simulink model "RobustFormationControl_IntegerModel"  (R2023a)
settings: Solver=ode3  StartTime=0.0  StopTime=30  FixedStep=0.0001  RelTol=1e-3
InitFcn:
  | % % Parameters for the fractional order NTFSMC:
  | % Sliding Surface " Sx, Sy, and Sz ":
  | %------------------------
  | % 10
  | % 10
  | cx = 2*[4 4 4];
  | cxx = 1*[0.01 0.01 0.01];
  | 
  | cx1 = cx(1);
  | cy1 = cx(2);
  | cz1 = cx(3);
  | 
  | cx2 = cxx(1);
  | cy2 = cxx(2);
  | cz2 = cxx(3);
  | 
  | alpha1 = [0.6 0.6 0.6];
  | alpha2 = [0.1 0.1 0.1];
  | 
  | gammaX = [3 3 3];
  | gx  = gammaX(1);
  | gy = gammaX(2);
  | gz = gammaX(3);
  | 
  | p = 10;
  | q = 10;
  | 
  | % Sliding Surface " S_Phi , S_Theta, and  S_Psi":
  | %------------------------
  | cP = 2*[4 4 4];
  | cPP = 1*[0.01 0.01 0.01 0.01];
  | 
  | cPhi1 = cP(1);
  | cTheta1 = cP(2);
  | cPsi1 = cP(3);
  | 
  | cPhi2 = cPP(1);
  | cTheta2 = cPP(2);
  | cPsi2 = cPP(3);
  | gammaP = [3 3 3];
  | 
  | %=========================
  | %=========================
  | SigmaX = 1*[0.01 0.01 0.01];
  | SigmaXX =1*[1 1 1];
  | 
  | Sigma1X = SigmaX(1);
  | Sigma1Y = SigmaX(2);
  | Sigma1Z = SigmaX(3);
  | %-----
  | Sigma2X = SigmaXX(1);
  | Sigma2Y = SigmaXX(2);
  | Sigma2Z = SigmaXX(3);
  | 
  | 
  | SigmaP = 1*[0.01 0.01 0.01];
  | SigmaPP =1*[1 1 1];
  | 
  | Sigma1Phi   = SigmaP(1);
  | Sigma1Theta = SigmaP(2);
  | ... (+80 lines)
values from neighbouring files (symbols this model uses):
  a1 = (Iyy - Izz)/Ixx    (= -0.812397034596)    [init_quadrotor_params.m]
  a2 = (Izz - Ixx)/Iyy    (= 0.812397034596)    [init_quadrotor_params.m]
  a3 = (Ixx - Iyy)/Izz    (= 0)    [init_quadrotor_params.m]
  a4 = - Ktx/m    (= -0.00114547325103)    [init_quadrotor_params.m]
  a5 = - Kty/m    (= -0.00114547325103)    [init_quadrotor_params.m]
  a6 = - Ktz/m    (= -0.00130740740741)    [init_quadrotor_params.m]
  b = 2.980e-5    (= 2.98e-05)    [init_quadrotor_params.m]
  b1 = - Jr/Ixx    (= -0.00584534596376)    [init_quadrotor_params.m]
  b2 = Jr/Iyy    (= 0.00584534596376)    [init_quadrotor_params.m]
  b3 = - Kfz/Izz    (= -0.0721963413248)    [init_quadrotor_params.m]
  b4 = 1/m    (= 2.05761316872)    [init_quadrotor_params.m]
  b5 = 1/m    (= 2.05761316872)    [init_quadrotor_params.m]
  b6 = 1/m    (= 2.05761316872)    [init_quadrotor_params.m]
  c1 = - Kfx/Ixx    (= -0.114641680395)    [init_quadrotor_params.m]
  c2 = - Kfy/Iyy    (= -0.114641680395)    [init_quadrotor_params.m]
  c3 = 1/Izz    (= 113.62345188)    [init_quadrotor_params.m]
  d = 1.12e-06    [init_quadrotor_params.m]
  d1 = L/Ixx    (= 46.334431631)    [init_quadrotor_params.m]
  d2 = L/Iyy    (= 46.334431631)    [init_quadrotor_params.m]
  g = 9.81    [init_quadrotor_params.m]
  Ixx = 4.856e-3    (= 0.004856)    [init_quadrotor_params.m]
  Iyy = 4.856e-3    (= 0.004856)    [init_quadrotor_params.m]
  Izz = 8.801e-3    (= 0.008801)    [init_quadrotor_params.m]
  Jr = 2.8385e-5    (= 2.8385e-05)    [init_quadrotor_params.m]
  Kfx = 5.567e-4    (= 0.0005567)    [init_quadrotor_params.m]
  Kfy = 5.567e-4    (= 0.0005567)    [init_quadrotor_params.m]
  Kfz = 6.354e-4    (= 0.0006354)    [init_quadrotor_params.m]
  Ktx = 5.5670e-4    (= 0.0005567)    [init_quadrotor_params.m]
  Kty = 5.5670e-4    (= 0.0005567)    [init_quadrotor_params.m]
  Ktz = 6.3540e-4    (= 0.0006354)    [init_quadrotor_params.m]
  L = 0.225    [init_quadrotor_params.m]
  m = 0.486    [init_quadrotor_params.m]
libraries: fod x120, eeStairGenerator x5
(part 4 of 9)

== system RobustFormationControl_IntegerModel/Integer Leader and four followers/Follower 1 System/Follower 1 Quadrotor Model/Quadrotor Dynamic System/Rotational System ==
  U2 : Inport
  U3 : Inport  Port=2
  U4 : Inport  Port=3
  Omega : Inport  Port=4
  Equation1 : Subsystem
  Equation2 : Subsystem
  Equation3 : Subsystem
  Phi or x1 : Outport  VectorParamsAs1DForOutWhenUnconnected=off
  Theta or x3 : Outport  Port=2  VectorParamsAs1DForOutWhenUnconnected=off
  Psi or x5 : Outport  Port=3  VectorParamsAs1DForOutWhenUnconnected=off
  x2 : Outport  Port=4  VectorParamsAs1DForOutWhenUnconnected=off
  x4 : Outport  Port=5  VectorParamsAs1DForOutWhenUnconnected=off
  x6 : Outport  Port=6  VectorParamsAs1DForOutWhenUnconnected=off
  wires:
  Equation1/1(x1 = Phi) -> Phi or x1/1
  Equation3/1(x5 =Psi) -> Psi or x5/1
  U2/1 -> Equation1/3(U2)
  U3/1 -> Equation2/3(U3)
  Equation3/2(x6) -> Equation2/2(x6), x6/1, Equation1/2(x6)
  Equation2/1(x3 =Theta) -> Theta or x3/1
  U4/1 -> Equation3/3(U4)
  Omega/1 -> Equation2/4(Omega), Equation1/4(Omega)
  Equation1/2(x2) -> x2/1, Equation2/1(x2), Equation3/1(x2)
  Equation2/2(x4) -> x4/1, Equation3/2(x4), Equation1/1(x4)

== system RobustFormationControl_IntegerModel/Integer Leader and four followers/Follower 1 System/Follower 1 Quadrotor Model/Quadrotor Dynamic System/Translational System ==
  U1 : Inport
  Ux : Inport  Port=2
  Uy : Inport  Port=3
  x1 : Inport  Port=4
  x3 : Inport  Port=5
  Equation4 : Subsystem
  Equation5 : Subsystem
  Equation6 : Subsystem
  x or x7 : Outport  VectorParamsAs1DForOutWhenUnconnected=off
  y or x9 : Outport  Port=2  VectorParamsAs1DForOutWhenUnconnected=off
  z or x11 : Outport  Port=3  VectorParamsAs1DForOutWhenUnconnected=off
  xdot or x8 : Outport  Port=4  VectorParamsAs1DForOutWhenUnconnected=off
  ydot or x10 : Outport  Port=5  VectorParamsAs1DForOutWhenUnconnected=off
  zdot or x12 : Outport  Port=6  VectorParamsAs1DForOutWhenUnconnected=off
  wires:
  Ux/1 -> Equation4/2(Ux)
  Uy/1 -> Equation5/2(Uy)
  x1/1 -> Equation6/2(x1)
  x3/1 -> Equation6/3(x3)
  Equation5/1(x9 = y) -> y or x9/1
  Equation6/1(x11 = z) -> z or x11/1
  Equation4/1(x7 = x) -> x or x7/1
  U1/1 -> Equation6/1(U1), Equation5/1(U1), Equation4/1(U1)
  Equation4/2(x8 = xdot) -> xdot or x8/1
  Equation5/2(x10 = ydot) -> ydot or x10/1
  Equation6/2(x12 = zdot) -> zdot or x12/1

== system RobustFormationControl_IntegerModel/Integer Leader and four followers/Follower 2 System/Follower 2 Quadrotor Model/Control Module1/Desired System ==
  Phi_d : Inport
  Theta_d : Inport  Port=2
  Psi_d : Inport  Port=3
  xd : Inport  Port=4
  yd : Inport  Port=5
  zd : Inport  Port=6
  Derivative{,1..5} (6 alike) : Derivative
  xd1 : Outport  VectorParamsAs1DForOutWhenUnconnected=off
  xd2 : Outport  Port=2  VectorParamsAs1DForOutWhenUnconnected=off
  xd3 : Outport  Port=3  VectorParamsAs1DForOutWhenUnconnected=off
  xd4 : Outport  Port=4  VectorParamsAs1DForOutWhenUnconnected=off
  xd5 : Outport  Port=5  VectorParamsAs1DForOutWhenUnconnected=off
  xd6 : Outport  Port=6  VectorParamsAs1DForOutWhenUnconnected=off
  xd7 : Outport  Port=7  VectorParamsAs1DForOutWhenUnconnected=off
  xd8 : Outport  Port=8  VectorParamsAs1DForOutWhenUnconnected=off
  xd9 : Outport  Port=9  VectorParamsAs1DForOutWhenUnconnected=off
  xd10 : Outport  Port=10  VectorParamsAs1DForOutWhenUnconnected=off
  xd11 : Outport  Port=11  VectorParamsAs1DForOutWhenUnconnected=off
  xd12 : Outport  Port=12  VectorParamsAs1DForOutWhenUnconnected=off
  wires:
  Phi_d/1 -> Derivative/1, xd1/1
  Derivative/1 -> xd2/1
  Derivative1/1 -> xd4/1
  Theta_d/1 -> Derivative1/1, xd3/1
  Psi_d/1 -> Derivative2/1, xd5/1
  Derivative2/1 -> xd6/1
  Derivative3/1 -> xd8/1
  Derivative4/1 -> xd10/1
  Derivative5/1 -> xd12/1
  xd/1 -> Derivative3/1, xd7/1
  yd/1 -> Derivative4/1, xd9/1
  zd/1 -> Derivative5/1, xd11/1

== system RobustFormationControl_IntegerModel/Integer Leader and four followers/Follower 2 System/Follower 2 Quadrotor Model/Control Module1/Omega Equations ==
  U1 : Inport
  U2 : Inport  Port=2
  U3 : Inport  Port=3
  U4 : Inport  Port=4
  Add1 : Sum  Inputs=+--
  Add2 : Sum  Inputs=+++
  Add3 : Sum  Inputs=++-
  Add5 : Sum  Inputs=+-+
  Control Inputs : Subsystem
  Gain11 : Gain  Gain=1/(4*b)
  Gain12 : Gain  Gain=1/(4*d)
  Gain7 : Gain  Gain=1/(2*b)
  Gain8 : Gain  Gain=1/(2*b)
  Omega : Outport  VectorParamsAs1DForOutWhenUnconnected=off
  wires:
  Add5/1 -> Control Inputs/1(w1_sqt)
  Add1/1 -> Control Inputs/2(w2_sqt)
  Add2/1 -> Control Inputs/3(w3_sqt)
  Gain11/1 -> Add5/1, Add3/1, Add2/1, Add1/1
  Gain12/1 -> Add5/3, Add2/3, Add3/3, Add1/3
  Gain7/1 -> Add5/2, Add2/2
  Gain8/1 -> Add3/2, Add1/2
  U4/1 -> Gain12/1
  U1/1 -> Gain11/1
  U3/1 -> Gain7/1
  U2/1 -> Gain8/1
  Add3/1 -> Control Inputs/4(w4_sqt)
  Control Inputs/1(Omega) -> Omega/1

== system RobustFormationControl_IntegerModel/Integer Leader and four followers/Follower 2 System/Follower 2 Quadrotor Model/Control Module1/Subsystem ==
  Ux : Inport
  Uy : Inport  Port=2
  Psi_d : Inport  Port=3
  Subsystem : Subsystem
  Subsystem1 : Subsystem
  Phi_d : Outport  VectorParamsAs1DForOutWhenUnconnected=off
  Theta_d : Outport  Port=2  VectorParamsAs1DForOutWhenUnconnected=off
  wires:
  Ux/1 -> Subsystem1/1(Ux), Subsystem/1(Ux)
  Uy/1 -> Subsystem1/2(Uy), Subsystem/2(Uy)
  Psi_d/1 -> Subsystem1/3(Psi_d), Subsystem/3(Psi_d)
  Subsystem/1(Phi_d) -> Subsystem1/4(Phi_d), Phi_d/1
  Subsystem1/1(Theta_d) -> Theta_d/1

== system RobustFormationControl_IntegerModel/Integer Leader and four followers/Follower 2 System/Follower 2 Quadrotor Model/Control Module1/Subsystem1 ==
  x1 : Inport
  x2 : Inport  Port=2
  x3 : Inport  Port=3
  x4 : Inport  Port=4
  x5 : Inport  Port=5
  x6 : Inport  Port=6
  x7 : Inport  Port=7
  x8 : Inport  Port=8
  x9 : Inport  Port=9
  x10 : Inport  Port=10
  x11 : Inport  Port=11
  x12 : Inport  Port=12
  xd1 : Inport  Port=13
  xd2 : Inport  Port=14
  xd3 : Inport  Port=15
  xd4 : Inport  Port=16
  xd5 : Inport  Port=17
  xd6 : Inport  Port=18
  xL : Inport  Port=19
  dX : Inport  Port=20
  yL : Inport  Port=21
  dY : Inport  Port=22
  zL : Inport  Port=23
  dZ : Inport  Port=24
  Subsystem : Subsystem
  Subsystem1 : Subsystem
  Subsystem2 : Subsystem
  Subsystem3 : Subsystem
  Subsystem4 : Subsystem
  Subsystem6 : Subsystem
  S2 : Outport  VectorParamsAs1DForOutWhenUnconnected=off
  S4 : Outport  Port=2  VectorParamsAs1DForOutWhenUnconnected=off
  S6 : Outport  Port=3  VectorParamsAs1DForOutWhenUnconnected=off
  S8 : Outport  Port=4  VectorParamsAs1DForOutWhenUnconnected=off
  S10 : Outport  Port=5  VectorParamsAs1DForOutWhenUnconnected=off
  S12 : Outport  Port=6  VectorParamsAs1DForOutWhenUnconnected=off
  wires:
  x1/1 -> [x1]
  x2/1 -> [x2]
  x3/1 -> [x3]
  x4/1 -> [x4]
  x5/1 -> [x5]
  x6/1 -> [x6]
  x7/1 -> [x7]
  x8/1 -> [x8]
  x9/1 -> [x9]
  x10/1 -> [x10]
  x11/1 -> [x11]
  x12/1 -> [x12]
  xd1/1 -> [xd1]
  dY/1 -> [dY]
  xd2/1 -> [xd2]
  xd3/1 -> [xd3]
  xd4/1 -> [xd4]
  xd5/1 -> [xd5]
  xd6/1 -> [xd6]
  xL/1 -> [xL]
  dX/1 -> [dX]
  yL/1 -> [yL]
  zL/1 -> [zL]
  dZ/1 -> [dZ]
  [x1] -> Subsystem/1(x1)
  [xd1] -> Subsystem/2(xd1)
  [x2] -> Subsystem/3(x2)
  [xd2] -> Subsystem/4(xd2)
  Subsystem/1(S2) -> S2/1
  [xd4] -> Subsystem6/4(xd4)
  [x3] -> Subsystem6/1(x3)
  [x4] -> Subsystem6/3(x4)
  [xd3] -> Subsystem6/2(xd3)
  [xd6] -> Subsystem1/4(xd6)
  [x5] -> Subsystem1/1(x5)
  [x6] -> Subsystem1/3(x6)
  [xd5] -> Subsystem1/2(xd5)
  Subsystem6/1(S4) -> S4/1
  Subsystem1/1(S6) -> S6/1
  [x9] -> Subsystem2/2(x9)
  [x10] -> Subsystem2/3(x10)
  [yL] -> Subsystem2/1(yL)
  [dY] -> Subsystem2/4(dY)
  Subsystem2/1(S10) -> S10/1
  [zL] -> Subsystem4/1(zL)
  [x8] -> Subsystem3/3(x8)
  Subsystem4/1(S12) -> S12/1
  [x12] -> Subsystem4/3(x12)
  Subsystem3/1(S8) -> S8/1
  [dZ] -> Subsystem4/4(dZ)
  [x11] -> Subsystem4/2(x11)
  [x7] -> Subsystem3/2(x7)
  [dX] -> Subsystem3/4(dX)
  [xL] -> Subsystem3/1(xL)

== system RobustFormationControl_IntegerModel/Integer Leader and four followers/Follower 2 System/Follower 2 Quadrotor Model/Control Module1/Subsystem10 ==
  x1 : Inport
  x3 : Inport  Port=2
  x11 : Inport  Port=3
  x12 : Inport  Port=4
  zL : Inport  Port=5
  dZ : Inport  Port=6
  S12 : Inport  Port=7
  Constant1 : Constant
  Divide1 : Product  Inputs=*/
  Divide2 : Product  Inputs=**  RndMeth=Zero  SaturateOnIntegerOverflow=on
  Gain : Gain  Commented=on  Gain=b6
  Product1 : Product
  Product2 : Product
  Subsystem : Subsystem
  Subsystem1 : Subsystem
  Subsystem2 : Subsystem
  Sum2 : Sum  Inputs=+++
  Trigonometric Function1 : Trigonometry  Operator=cos
  Trigonometric Function2 : Trigonometry  Operator=cos
  U1 : Outport  VectorParamsAs1DForOutWhenUnconnected=off
  wires:
  S12/1 -> [S12]
  dZ/1 -> [dZ]
  zL/1 -> [zL]
  x3/1 -> [x3]
  Sum2/1 -> Product2/2
  Product2/1 -> U1/1
  x11/1 -> [x11]
  x12/1 -> [x12]
  x1/1 -> [x1]
  [x11] -> Subsystem/2(x11)
  [x12] -> Subsystem1/1(x12)
  [zL] -> Subsystem1/2(zL)
  [zL] -> Subsystem/1(zL)
  [dZ] -> Subsystem/4(dZ)
  [x12] -> Subsystem/3(x12)
  [S12] -> Subsystem/5(S12)
  [x11] -> Subsystem2/2(x11)
  [S12] -> Subsystem2/5(S12)
  [x12] -> Subsystem2/3(x12)
  [zL] -> Subsystem2/1(zL)
  [dZ] -> Subsystem2/4(dZ)
  Subsystem/1(D2) -> Sum2/2
  Subsystem2/1(D3) -> Sum2/3
  Subsystem1/1(D1) -> Sum2/1
  Divide1/1 -> Product2/1
  Constant1/1 -> Divide1/1
  Trigonometric Function2/1 -> Product1/2
  Trigonometric Function1/1 -> Product1/1
  Divide2/1 -> Divide1/2
  Product1/1 -> Divide2/2
  [x1] -> Trigonometric Function1/1
  [x3] -> Trigonometric Function2/1
  [b6D] -> Divide2/1
  [dZ] -> Subsystem1/3(dZ)

== system RobustFormationControl_IntegerModel/Integer Leader and four followers/Follower 2 System/Follower 2 Quadrotor Model/Control Module1/Subsystem2 ==
  U1 : Inport
  x9 : Inport  Port=2
  x10 : Inport  Port=3
  yL : Inport  Port=4
  dY : Inport  Port=5
  S10 : Inport  Port=6
  Constant1 : Constant
  Divide1 : Product  Inputs=*/
  Divide2 : Product  Inputs=**  RndMeth=Zero  SaturateOnIntegerOverflow=on
  Gain1 : Gain  Commented=on  Gain=b4
  Product2 : Product
  Subsystem3 : Subsystem
  Subsystem4 : Subsystem
  Subsystem5 : Subsystem
  Sum1 : Sum  Inputs=+++
  Uy : Outport  VectorParamsAs1DForOutWhenUnconnected=off
  wires:
  S10/1 -> [S10]
  dY/1 -> [dY]
  yL/1 -> [yL]
  Product2/1 -> Uy/1
  x9/1 -> [x9]
  x10/1 -> [x10]
  U1/1 -> [U1]
  Divide1/1 -> Product2/1
  Constant1/1 -> Divide1/1
  [b5D] -> Divide2/1
  [U1] -> Divide2/2
  Divide2/1 -> Divide1/2
  [dY] -> Subsystem4/3(dY)
  [dY] -> Subsystem3/4(dY)
  Subsystem4/1(D1) -> Sum1/1
  Subsystem5/1(D3) -> Sum1/3
  [yL] -> Subsystem5/1(yL)
  Subsystem3/1(D2) -> Sum1/2
  [dY] -> Subsystem5/4(dY)
  [x9] -> Subsystem3/2(x9)
  [yL] -> Subsystem3/1(yL)
  [yL] -> Subsystem4/2(yL)
  [S10] -> Subsystem3/5(S10)
  [x9] -> Subsystem5/2(x9)
  [x10] -> Subsystem5/3(x10)
  [x10] -> Subsystem4/1(x10)
  [x10] -> Subsystem3/3(x10)
  [S10] -> Subsystem5/5(S10)
  Sum1/1 -> Product2/2

== system RobustFormationControl_IntegerModel/Integer Leader and four followers/Follower 2 System/Follower 2 Quadrotor Model/Control Module1/Subsystem4 ==
  x1 : Inport
  x2 : Inport  Port=2
  x4 : Inport  Port=3
  x6 : Inport  Port=4
  xd1 : Inport  Port=5
  xd2 : Inport  Port=6
  S2 : Inport  Port=7
  Omega : Inport  Port=8
  Constant : Constant
  Constant3 : Constant  Value=d1
  Derivative : Derivative
  Divide : Product  Inputs=*/
  Product2 : Product
  Subsystem : Subsystem
  Subsystem1 : Subsystem
  Subsystem2 : Subsystem
  Sum2 : Sum  Inputs=+++
  U2 : Outport  VectorParamsAs1DForOutWhenUnconnected=off
  wires:
  Constant/1 -> Divide/1
  Constant3/1 -> Divide/2
  S2/1 -> [S2]
  xd2/1 -> [xd2], Derivative/1
  Derivative/1 -> [xdDot2]
  xd1/1 -> [xd1]
  x2/1 -> [x2]
  Sum2/1 -> Product2/2
  Divide/1 -> Product2/1
  Product2/1 -> U2/1
  x4/1 -> [x4]
  x6/1 -> [x6]
  x1/1 -> [x1]
  [x1] -> Subsystem/1(x1)
  [x4] -> Subsystem1/1(x4)
  [x6] -> Subsystem1/2(x6)
  [x2] -> Subsystem1/3(x2)
  Omega/1 -> Subsystem1/4(Omega)
  [xdDot2] -> Subsystem1/5(xd2)
  [xd1] -> Subsystem/2(xd1)
  [xd2] -> Subsystem/4(xd2)
  [x2] -> Subsystem/3(x2)
  [S2] -> Subsystem/5(S2)
  [xd1] -> Subsystem2/2(xd1)
  [S2] -> Subsystem2/5(S2)
  [x2] -> Subsystem2/3(x2)
  [x1] -> Subsystem2/1(x1)
  [xd2] -> Subsystem2/4(xd2)
  Subsystem1/1(D1) -> Sum2/1
  Subsystem/1(D2) -> Sum2/2
  Subsystem2/1(D3) -> Sum2/3

== system RobustFormationControl_IntegerModel/Integer Leader and four followers/Follower 2 System/Follower 2 Quadrotor Model/Control Module1/Subsystem5 ==
  x5 : Inport
  x2 : Inport  Port=2
  x4 : Inport  Port=3
  x6 : Inport  Port=4
  xd5 : Inport  Port=5
  xd6 : Inport  Port=6
  S6 : Inport  Port=7
  Constant : Constant
  Constant3 : Constant  Value=c3
  Derivative : Derivative
  Divide : Product  Inputs=*/
  Product2 : Product
  Subsystem : Subsystem
  Subsystem1 : Subsystem
  Subsystem2 : Subsystem
  Sum2 : Sum  Inputs=+++
  U4 : Outport  VectorParamsAs1DForOutWhenUnconnected=off
  wires:
  Constant/1 -> Divide/1
  Constant3/1 -> Divide/2
  S6/1 -> [S6]
  xd6/1 -> [xd6], Derivative/1
  Derivative/1 -> [xdDot6]
  xd5/1 -> [xd5]
  x2/1 -> [x2]
  Sum2/1 -> Product2/2
  Divide/1 -> Product2/1
  Product2/1 -> U4/1
  x4/1 -> [x4]
  x6/1 -> [x6]
  x5/1 -> [x5]
  [x5] -> Subsystem/1(x5)
  [x4] -> Subsystem1/1(x4)
  [x6] -> Subsystem1/2(x6)
  [x2] -> Subsystem1/3(x2)
  [xdDot6] -> Subsystem1/4(xd6)
  [xd5] -> Subsystem/2(xd5)
  [xd6] -> Subsystem/4(xd6)
  [x6] -> Subsystem/3(x6)
  [S6] -> Subsystem/5(S4)
  [xd5] -> Subsystem2/2(xd5)
  [S6] -> Subsystem2/5(S6)
  [x6] -> Subsystem2/3(x6)
  [x5] -> Subsystem2/1(x5)
  [xd6] -> Subsystem2/4(xd6)
  Subsystem/1(D2) -> Sum2/2
  Subsystem2/1(D3) -> Sum2/3
  Subsystem1/1(D1) -> Sum2/1

== system RobustFormationControl_IntegerModel/Integer Leader and four followers/Follower 2 System/Follower 2 Quadrotor Model/Control Module1/Subsystem6 ==
  U1 : Inport
  x7 : Inport  Port=2
  x8 : Inport  Port=3
  xL : Inport  Port=4
  dX : Inport  Port=5
  S8 : Inport  Port=6
  Constant1 : Constant
  Divide1 : Product  Inputs=*/
  Divide2 : Product  Inputs=**  RndMeth=Zero  SaturateOnIntegerOverflow=on
  Gain1 : Gain  Commented=on  Gain=b4
  Product2 : Product
  Subsystem3 : Subsystem
  Subsystem4 : Subsystem
  Subsystem5 : Subsystem
  Sum1 : Sum  Inputs=+++
  Ux : Outport  VectorParamsAs1DForOutWhenUnconnected=off
  wires:
  S8/1 -> [S8]
  dX/1 -> [dX]
  xL/1 -> [xL]
  Product2/1 -> Ux/1
  x7/1 -> [x7]
  x8/1 -> [x8]
  U1/1 -> [U1]
  Divide1/1 -> Product2/1
  Constant1/1 -> Divide1/1
  [b4D] -> Divide2/1
  [U1] -> Divide2/2
  Divide2/1 -> Divide1/2
  [dX] -> Subsystem4/3(dX)
  [dX] -> Subsystem3/4(dX)
  Subsystem4/1(D1) -> Sum1/1
  Subsystem5/1(D3) -> Sum1/3
  [xL] -> Subsystem5/1(xL)
  Subsystem3/1(D2) -> Sum1/2
  [dX] -> Subsystem5/4(dX)
  [x7] -> Subsystem3/2(x7)
  [xL] -> Subsystem3/1(xL)
  [xL] -> Subsystem4/2(xL)
  [S8] -> Subsystem3/5(S8)
  [x7] -> Subsystem5/2(x7)
  [x8] -> Subsystem5/3(x8)
  [x8] -> Subsystem4/1(x8)
  [x8] -> Subsystem3/3(x8)
  [S8] -> Subsystem5/5(S8)
  Sum1/1 -> Product2/2

== system RobustFormationControl_IntegerModel/Integer Leader and four followers/Follower 2 System/Follower 2 Quadrotor Model/Control Module1/Subsystem8 ==
  x3 : Inport
  x2 : Inport  Port=2
  x4 : Inport  Port=3
  x6 : Inport  Port=4
  xd3 : Inport  Port=5
  xd4 : Inport  Port=6
  S4 : Inport  Port=7
  Omega : Inport  Port=8
  Constant : Constant
  Constant3 : Constant  Value=d2
  Derivative : Derivative
  Divide : Product  Inputs=*/
  Product2 : Product
  Subsystem : Subsystem
  Subsystem1 : Subsystem
  Subsystem2 : Subsystem
  Sum2 : Sum  Inputs=+++
  U3 : Outport  VectorParamsAs1DForOutWhenUnconnected=off
  wires:
  Constant/1 -> Divide/1
  Constant3/1 -> Divide/2
  S4/1 -> [S4]
  xd4/1 -> [xd4], Derivative/1
  Derivative/1 -> [xdDot4]
  xd3/1 -> [xd3]
  x2/1 -> [x2]
  Sum2/1 -> Product2/2
  Divide/1 -> Product2/1
  Product2/1 -> U3/1
  x4/1 -> [x4]
  x6/1 -> [x6]
  x3/1 -> [x3]
  [x3] -> Subsystem/1(x3)
  [x4] -> Subsystem1/1(x4)
  [x6] -> Subsystem1/2(x6)
  [x2] -> Subsystem1/3(x2)
  Omega/1 -> Subsystem1/4(Omega)
  [xdDot4] -> Subsystem1/5(xd4)
  [xd3] -> Subsystem/2(xd3)
  [xd4] -> Subsystem/4(xd4)
  [x4] -> Subsystem/3(x4)
  [S4] -> Subsystem/5(S4)
  [xd3] -> Subsystem2/2(xd3)
  [S4] -> Subsystem2/5(S4)
  [x4] -> Subsystem2/3(x4)
  [x3] -> Subsystem2/1(x3)
  [xd4] -> Subsystem2/4(xd4)
  Subsystem/1(D2) -> Sum2/2
  Subsystem2/1(D3) -> Sum2/3
  Subsystem1/1(D1) -> Sum2/1

== system RobustFormationControl_IntegerModel/Integer Leader and four followers/Follower 2 System/Follower 2 Quadrotor Model/Quadrotor Dynamic System/Rotational System ==
  U2 : Inport
  U3 : Inport  Port=2
  U4 : Inport  Port=3
  Omega : Inport  Port=4
  Equation1 : Subsystem
  Equation2 : Subsystem
  Equation3 : Subsystem
  Phi or x1 : Outport  VectorParamsAs1DForOutWhenUnconnected=off
  Theta or x3 : Outport  Port=2  VectorParamsAs1DForOutWhenUnconnected=off
  Psi or x5 : Outport  Port=3  VectorParamsAs1DForOutWhenUnconnected=off
  x2 : Outport  Port=4  VectorParamsAs1DForOutWhenUnconnected=off
  x4 : Outport  Port=5  VectorParamsAs1DForOutWhenUnconnected=off
  x6 : Outport  Port=6  VectorParamsAs1DForOutWhenUnconnected=off
  wires:
  Equation1/1(x1 = Phi) -> Phi or x1/1
  Equation3/1(x5 =Psi) -> Psi or x5/1
  U2/1 -> Equation1/3(U2)
  U3/1 -> Equation2/3(U3)
  Equation3/2(x6) -> Equation2/2(x6), x6/1, Equation1/2(x6)
  Equation2/1(x3 =Theta) -> Theta or x3/1
  U4/1 -> Equation3/3(U4)
  Omega/1 -> Equation2/4(Omega), Equation1/4(Omega)
  Equation1/2(x2) -> x2/1, Equation2/1(x2), Equation3/1(x2)
  Equation2/2(x4) -> x4/1, Equation3/2(x4), Equation1/1(x4)

== system RobustFormationControl_IntegerModel/Integer Leader and four followers/Follower 2 System/Follower 2 Quadrotor Model/Quadrotor Dynamic System/Translational System ==
  U1 : Inport
  Ux : Inport  Port=2
  Uy : Inport  Port=3
  x1 : Inport  Port=4
  x3 : Inport  Port=5
  Equation4 : Subsystem
  Equation5 : Subsystem
  Equation6 : Subsystem
  x or x7 : Outport  VectorParamsAs1DForOutWhenUnconnected=off
  y or x9 : Outport  Port=2  VectorParamsAs1DForOutWhenUnconnected=off
  z or x11 : Outport  Port=3  VectorParamsAs1DForOutWhenUnconnected=off
  xdot or x8 : Outport  Port=4  VectorParamsAs1DForOutWhenUnconnected=off
  ydot or x10 : Outport  Port=5  VectorParamsAs1DForOutWhenUnconnected=off
  zdot or x12 : Outport  Port=6  VectorParamsAs1DForOutWhenUnconnected=off
  wires:
  Ux/1 -> Equation4/2(Ux)
  Uy/1 -> Equation5/2(Uy)
  x1/1 -> Equation6/2(x1)
  x3/1 -> Equation6/3(x3)
  Equation5/1(x9 = y) -> y or x9/1
  Equation6/1(x11 = z) -> z or x11/1
  Equation4/1(x7 = x) -> x or x7/1
  U1/1 -> Equation6/1(U1), Equation5/1(U1), Equation4/1(U1)
  Equation4/2(x8 = xdot) -> xdot or x8/1
  Equation5/2(x10 = ydot) -> ydot or x10/1
  Equation6/2(x12 = zdot) -> zdot or x12/1

== system RobustFormationControl_IntegerModel/Integer Leader and four followers/Follower 3 System/Follower 2 Quadrotor Model/Control Module1/Desired System ==
  Phi_d : Inport
  Theta_d : Inport  Port=2
  Psi_d : Inport  Port=3
  xd : Inport  Port=4
  yd : Inport  Port=5
  zd : Inport  Port=6
  Derivative{,1..5} (6 alike) : Derivative
  xd1 : Outport  VectorParamsAs1DForOutWhenUnconnected=off
  xd2 : Outport  Port=2  VectorParamsAs1DForOutWhenUnconnected=off
  xd3 : Outport  Port=3  VectorParamsAs1DForOutWhenUnconnected=off
  xd4 : Outport  Port=4  VectorParamsAs1DForOutWhenUnconnected=off
  xd5 : Outport  Port=5  VectorParamsAs1DForOutWhenUnconnected=off
  xd6 : Outport  Port=6  VectorParamsAs1DForOutWhenUnconnected=off
  xd7 : Outport  Port=7  VectorParamsAs1DForOutWhenUnconnected=off
  xd8 : Outport  Port=8  VectorParamsAs1DForOutWhenUnconnected=off
  xd9 : Outport  Port=9  VectorParamsAs1DForOutWhenUnconnected=off
  xd10 : Outport  Port=10  VectorParamsAs1DForOutWhenUnconnected=off
  xd11 : Outport  Port=11  VectorParamsAs1DForOutWhenUnconnected=off
  xd12 : Outport  Port=12  VectorParamsAs1DForOutWhenUnconnected=off
  wires:
  zd/1 -> xd11/1, Derivative5/1
  yd/1 -> xd9/1, Derivative4/1
  xd/1 -> xd7/1, Derivative3/1
  Derivative5/1 -> xd12/1
  Derivative4/1 -> xd10/1
  Derivative3/1 -> xd8/1
  Derivative2/1 -> xd6/1
  Psi_d/1 -> xd5/1, Derivative2/1
  Theta_d/1 -> xd3/1, Derivative1/1
  Derivative1/1 -> xd4/1
  Derivative/1 -> xd2/1
  Phi_d/1 -> xd1/1, Derivative/1

== system RobustFormationControl_IntegerModel/Integer Leader and four followers/Follower 3 System/Follower 2 Quadrotor Model/Control Module1/Omega Equations ==
  U1 : Inport
  U2 : Inport  Port=2
  U3 : Inport  Port=3
  U4 : Inport  Port=4
  Add1 : Sum  Inputs=+--
  Add2 : Sum  Inputs=+++
  Add3 : Sum  Inputs=++-
  Add5 : Sum  Inputs=+-+
  Control Inputs : Subsystem
  Gain11 : Gain  Gain=1/(4*b)
  Gain12 : Gain  Gain=1/(4*d)
  Gain7 : Gain  Gain=1/(2*b)
  Gain8 : Gain  Gain=1/(2*b)
  Omega : Outport  VectorParamsAs1DForOutWhenUnconnected=off
  wires:
  Control Inputs/1(Omega) -> Omega/1
  Add3/1 -> Control Inputs/4(w4_sqt)
  U2/1 -> Gain8/1
  U3/1 -> Gain7/1
  U1/1 -> Gain11/1
  U4/1 -> Gain12/1
  Gain8/1 -> Add1/2, Add3/2
  Gain7/1 -> Add2/2, Add5/2
  Gain12/1 -> Add1/3, Add3/3, Add2/3, Add5/3
  Gain11/1 -> Add1/1, Add2/1, Add3/1, Add5/1
  Add2/1 -> Control Inputs/3(w3_sqt)
  Add1/1 -> Control Inputs/2(w2_sqt)
  Add5/1 -> Control Inputs/1(w1_sqt)

== system RobustFormationControl_IntegerModel/Integer Leader and four followers/Follower 3 System/Follower 2 Quadrotor Model/Control Module1/Subsystem ==
  Ux : Inport
  Uy : Inport  Port=2
  Psi_d : Inport  Port=3
  Subsystem : Subsystem
  Subsystem1 : Subsystem
  Phi_d : Outport  VectorParamsAs1DForOutWhenUnconnected=off
  Theta_d : Outport  Port=2  VectorParamsAs1DForOutWhenUnconnected=off
  wires:
  Subsystem1/1(Theta_d) -> Theta_d/1
  Subsystem/1(Phi_d) -> Phi_d/1, Subsystem1/4(Phi_d)
  Psi_d/1 -> Subsystem/3(Psi_d), Subsystem1/3(Psi_d)
  Uy/1 -> Subsystem/2(Uy), Subsystem1/2(Uy)
  Ux/1 -> Subsystem/1(Ux), Subsystem1/1(Ux)

== system RobustFormationControl_IntegerModel/Integer Leader and four followers/Follower 3 System/Follower 2 Quadrotor Model/Control Module1/Subsystem1 ==
  x1 : Inport
  x2 : Inport  Port=2
  x3 : Inport  Port=3
  x4 : Inport  Port=4
  x5 : Inport  Port=5
  x6 : Inport  Port=6
  x7 : Inport  Port=7
  x8 : Inport  Port=8
  x9 : Inport  Port=9
  x10 : Inport  Port=10
  x11 : Inport  Port=11
  x12 : Inport  Port=12
  xd1 : Inport  Port=13
  xd2 : Inport  Port=14
  xd3 : Inport  Port=15
  xd4 : Inport  Port=16
  xd5 : Inport  Port=17
  xd6 : Inport  Port=18
  xL : Inport  Port=19
  dX : Inport  Port=20
  yL : Inport  Port=21
  dY : Inport  Port=22
  zL : Inport  Port=23
  dZ : Inport  Port=24
  Subsystem : Subsystem
  Subsystem1 : Subsystem
  Subsystem2 : Subsystem
  Subsystem3 : Subsystem
  Subsystem4 : Subsystem
  Subsystem6 : Subsystem
  S2 : Outport  VectorParamsAs1DForOutWhenUnconnected=off
  S4 : Outport  Port=2  VectorParamsAs1DForOutWhenUnconnected=off
  S6 : Outport  Port=3  VectorParamsAs1DForOutWhenUnconnected=off
  S8 : Outport  Port=4  VectorParamsAs1DForOutWhenUnconnected=off
  S10 : Outport  Port=5  VectorParamsAs1DForOutWhenUnconnected=off
  S12 : Outport  Port=6  VectorParamsAs1DForOutWhenUnconnected=off
  wires:
  [xL] -> Subsystem3/1(xL)
  [dX] -> Subsystem3/4(dX)
  [x7] -> Subsystem3/2(x7)
  [x11] -> Subsystem4/2(x11)
  [dZ] -> Subsystem4/4(dZ)
  Subsystem3/1(S8) -> S8/1
  [x12] -> Subsystem4/3(x12)
  Subsystem4/1(S12) -> S12/1
  [x8] -> Subsystem3/3(x8)
  [zL] -> Subsystem4/1(zL)
  Subsystem2/1(S10) -> S10/1
  [dY] -> Subsystem2/4(dY)
  [yL] -> Subsystem2/1(yL)
  [x10] -> Subsystem2/3(x10)
  [x9] -> Subsystem2/2(x9)
  Subsystem1/1(S6) -> S6/1
  Subsystem6/1(S4) -> S4/1
  [xd5] -> Subsystem1/2(xd5)
  [x6] -> Subsystem1/3(x6)
  [x5] -> Subsystem1/1(x5)
  [xd6] -> Subsystem1/4(xd6)
  [xd3] -> Subsystem6/2(xd3)
  [x4] -> Subsystem6/3(x4)
  [x3] -> Subsystem6/1(x3)
  [xd4] -> Subsystem6/4(xd4)
  Subsystem/1(S2) -> S2/1
  [xd2] -> Subsystem/4(xd2)
  [x2] -> Subsystem/3(x2)
  [xd1] -> Subsystem/2(xd1)
  [x1] -> Subsystem/1(x1)
  dZ/1 -> [dZ]
  zL/1 -> [zL]
  yL/1 -> [yL]
  dX/1 -> [dX]
  xL/1 -> [xL]
  xd6/1 -> [xd6]
  xd5/1 -> [xd5]
  xd4/1 -> [xd4]
  xd3/1 -> [xd3]
  xd2/1 -> [xd2]
  dY/1 -> [dY]
  xd1/1 -> [xd1]
  x12/1 -> [x12]
  x11/1 -> [x11]
  x10/1 -> [x10]
  x9/1 -> [x9]
  x8/1 -> [x8]
  x7/1 -> [x7]
  x6/1 -> [x6]
  x5/1 -> [x5]
  x4/1 -> [x4]
  x3/1 -> [x3]
  x2/1 -> [x2]
  x1/1 -> [x1]

== system RobustFormationControl_IntegerModel/Integer Leader and four followers/Follower 3 System/Follower 2 Quadrotor Model/Control Module1/Subsystem10 ==
  x1 : Inport
  x3 : Inport  Port=2
  x11 : Inport  Port=3
  x12 : Inport  Port=4
  zL : Inport  Port=5
  dZ : Inport  Port=6
  S12 : Inport  Port=7
  Constant1 : Constant
  Divide1 : Product  Inputs=*/
  Divide2 : Product  Inputs=**  RndMeth=Zero  SaturateOnIntegerOverflow=on
  Gain : Gain  Commented=on  Gain=b6
  Product1 : Product
  Product2 : Product
  Subsystem : Subsystem
  Subsystem1 : Subsystem
  Subsystem2 : Subsystem
  Sum2 : Sum  Inputs=+++
  Trigonometric Function1 : Trigonometry  Operator=cos
  Trigonometric Function2 : Trigonometry  Operator=cos
  U1 : Outport  VectorParamsAs1DForOutWhenUnconnected=off
  wires:
  [dZ] -> Subsystem1/3(dZ)
  [b6D] -> Divide2/1
  [x3] -> Trigonometric Function2/1
  [x1] -> Trigonometric Function1/1
  Product1/1 -> Divide2/2
  Divide2/1 -> Divide1/2
  Trigonometric Function1/1 -> Product1/1
  Trigonometric Function2/1 -> Product1/2
  Constant1/1 -> Divide1/1
  Divide1/1 -> Product2/1
  Subsystem1/1(D1) -> Sum2/1
  Subsystem2/1(D3) -> Sum2/3
  Subsystem/1(D2) -> Sum2/2
  [dZ] -> Subsystem2/4(dZ)
  [zL] -> Subsystem2/1(zL)
  [x12] -> Subsystem2/3(x12)
  [S12] -> Subsystem2/5(S12)
  [x11] -> Subsystem2/2(x11)
  [S12] -> Subsystem/5(S12)
  [x12] -> Subsystem/3(x12)
  [dZ] -> Subsystem/4(dZ)
  [zL] -> Subsystem/1(zL)
  [zL] -> Subsystem1/2(zL)
  [x12] -> Subsystem1/1(x12)
  [x11] -> Subsystem/2(x11)
  x1/1 -> [x1]
  x12/1 -> [x12]
  x11/1 -> [x11]
  Product2/1 -> U1/1
  Sum2/1 -> Product2/2
  x3/1 -> [x3]
  zL/1 -> [zL]
  dZ/1 -> [dZ]
  S12/1 -> [S12]

== system RobustFormationControl_IntegerModel/Integer Leader and four followers/Follower 3 System/Follower 2 Quadrotor Model/Control Module1/Subsystem2 ==
  U1 : Inport
  x9 : Inport  Port=2
  x10 : Inport  Port=3
  yL : Inport  Port=4
  dY : Inport  Port=5
  S10 : Inport  Port=6
  Constant1 : Constant
  Divide1 : Product  Inputs=*/
  Divide2 : Product  Inputs=**  RndMeth=Zero  SaturateOnIntegerOverflow=on
  Gain1 : Gain  Commented=on  Gain=b4
  Product2 : Product
  Subsystem3 : Subsystem
  Subsystem4 : Subsystem
  Subsystem5 : Subsystem
  Sum1 : Sum  Inputs=+++
  Uy : Outport  VectorParamsAs1DForOutWhenUnconnected=off
  wires:
  Sum1/1 -> Product2/2
  [S10] -> Subsystem5/5(S10)
  [x10] -> Subsystem3/3(x10)
  [x10] -> Subsystem4/1(x10)
  [x10] -> Subsystem5/3(x10)
  [x9] -> Subsystem5/2(x9)
  [S10] -> Subsystem3/5(S10)
  [yL] -> Subsystem4/2(yL)
  [yL] -> Subsystem3/1(yL)
  [x9] -> Subsystem3/2(x9)
  [dY] -> Subsystem5/4(dY)
  Subsystem3/1(D2) -> Sum1/2
  [yL] -> Subsystem5/1(yL)
  Subsystem5/1(D3) -> Sum1/3
  Subsystem4/1(D1) -> Sum1/1
  [dY] -> Subsystem3/4(dY)
  [dY] -> Subsystem4/3(dY)
  Divide2/1 -> Divide1/2
  [U1] -> Divide2/2
  [b5D] -> Divide2/1
  Constant1/1 -> Divide1/1
  Divide1/1 -> Product2/1
  U1/1 -> [U1]
  x10/1 -> [x10]
  x9/1 -> [x9]
  Product2/1 -> Uy/1
  yL/1 -> [yL]
  dY/1 -> [dY]
  S10/1 -> [S10]

== system RobustFormationControl_IntegerModel/Integer Leader and four followers/Follower 3 System/Follower 2 Quadrotor Model/Control Module1/Subsystem4 ==
  x1 : Inport
  x2 : Inport  Port=2
  x4 : Inport  Port=3
  x6 : Inport  Port=4
  xd1 : Inport  Port=5
  xd2 : Inport  Port=6
  S2 : Inport  Port=7
  Omega : Inport  Port=8
  Constant : Constant
  Constant3 : Constant  Value=d1
  Derivative : Derivative
  Divide : Product  Inputs=*/
  Product2 : Product
  Subsystem : Subsystem
  Subsystem1 : Subsystem
  Subsystem2 : Subsystem
  Sum2 : Sum  Inputs=+++
  U2 : Outport  VectorParamsAs1DForOutWhenUnconnected=off
  wires:
  Subsystem2/1(D3) -> Sum2/3
  Subsystem/1(D2) -> Sum2/2
  Subsystem1/1(D1) -> Sum2/1
  [xd2] -> Subsystem2/4(xd2)
  [x1] -> Subsystem2/1(x1)
  [x2] -> Subsystem2/3(x2)
  [S2] -> Subsystem2/5(S2)
  [xd1] -> Subsystem2/2(xd1)
  [S2] -> Subsystem/5(S2)
  [x2] -> Subsystem/3(x2)
  [xd2] -> Subsystem/4(xd2)
  [xd1] -> Subsystem/2(xd1)
  [xdDot2] -> Subsystem1/5(xd2)
  Omega/1 -> Subsystem1/4(Omega)
  [x2] -> Subsystem1/3(x2)
  [x6] -> Subsystem1/2(x6)
  [x4] -> Subsystem1/1(x4)
  [x1] -> Subsystem/1(x1)
  x1/1 -> [x1]
  x6/1 -> [x6]
  x4/1 -> [x4]
  Product2/1 -> U2/1
  Divide/1 -> Product2/1
  Sum2/1 -> Product2/2
  x2/1 -> [x2]
  xd1/1 -> [xd1]
  Derivative/1 -> [xdDot2]
  xd2/1 -> Derivative/1, [xd2]
  S2/1 -> [S2]
  Constant3/1 -> Divide/2
  Constant/1 -> Divide/1

== system RobustFormationControl_IntegerModel/Integer Leader and four followers/Follower 3 System/Follower 2 Quadrotor Model/Control Module1/Subsystem5 ==
  x5 : Inport
  x2 : Inport  Port=2
  x4 : Inport  Port=3
  x6 : Inport  Port=4
  xd5 : Inport  Port=5
  xd6 : Inport  Port=6
  S6 : Inport  Port=7
  Constant : Constant
  Constant3 : Constant  Value=c3
  Derivative : Derivative
  Divide : Product  Inputs=*/
  Product2 : Product
  Subsystem : Subsystem
  Subsystem1 : Subsystem
  Subsystem2 : Subsystem
  Sum2 : Sum  Inputs=+++
  U4 : Outport  VectorParamsAs1DForOutWhenUnconnected=off
  wires:
  Subsystem1/1(D1) -> Sum2/1
  Subsystem2/1(D3) -> Sum2/3
  Subsystem/1(D2) -> Sum2/2
  [xd6] -> Subsystem2/4(xd6)
  [x5] -> Subsystem2/1(x5)
  [x6] -> Subsystem2/3(x6)
  [S6] -> Subsystem2/5(S6)
  [xd5] -> Subsystem2/2(xd5)
  [S6] -> Subsystem/5(S4)
  [x6] -> Subsystem/3(x6)
  [xd6] -> Subsystem/4(xd6)
  [xd5] -> Subsystem/2(xd5)
  [xdDot6] -> Subsystem1/4(xd6)
  [x2] -> Subsystem1/3(x2)
  [x6] -> Subsystem1/2(x6)
  [x4] -> Subsystem1/1(x4)
  [x5] -> Subsystem/1(x5)
  x5/1 -> [x5]
  x6/1 -> [x6]
  x4/1 -> [x4]
  Product2/1 -> U4/1
  Divide/1 -> Product2/1
  Sum2/1 -> Product2/2
  x2/1 -> [x2]
  xd5/1 -> [xd5]
  Derivative/1 -> [xdDot6]
  xd6/1 -> Derivative/1, [xd6]
  S6/1 -> [S6]
  Constant3/1 -> Divide/2
  Constant/1 -> Divide/1

== system RobustFormationControl_IntegerModel/Integer Leader and four followers/Follower 3 System/Follower 2 Quadrotor Model/Control Module1/Subsystem6 ==
  U1 : Inport
  x7 : Inport  Port=2
  x8 : Inport  Port=3
  xL : Inport  Port=4
  dX : Inport  Port=5
  S8 : Inport  Port=6
  Constant1 : Constant
  Divide1 : Product  Inputs=*/
  Divide2 : Product  Inputs=**  RndMeth=Zero  SaturateOnIntegerOverflow=on
  Gain1 : Gain  Commented=on  Gain=b4
  Product2 : Product
  Subsystem3 : Subsystem
  Subsystem4 : Subsystem
  Subsystem5 : Subsystem
  Sum1 : Sum  Inputs=+++
  Ux : Outport  VectorParamsAs1DForOutWhenUnconnected=off
  wires:
  Sum1/1 -> Product2/2
  [S8] -> Subsystem5/5(S8)
  [x8] -> Subsystem3/3(x8)
  [x8] -> Subsystem4/1(x8)
  [x8] -> Subsystem5/3(x8)
  [x7] -> Subsystem5/2(x7)
  [S8] -> Subsystem3/5(S8)
  [xL] -> Subsystem4/2(xL)
  [xL] -> Subsystem3/1(xL)
  [x7] -> Subsystem3/2(x7)
  [dX] -> Subsystem5/4(dX)
  Subsystem3/1(D2) -> Sum1/2
  [xL] -> Subsystem5/1(xL)
  Subsystem5/1(D3) -> Sum1/3
  Subsystem4/1(D1) -> Sum1/1
  [dX] -> Subsystem3/4(dX)
  [dX] -> Subsystem4/3(dX)
  Divide2/1 -> Divide1/2
  [U1] -> Divide2/2
  [b4D] -> Divide2/1
  Constant1/1 -> Divide1/1
  Divide1/1 -> Product2/1
  U1/1 -> [U1]
  x8/1 -> [x8]
  x7/1 -> [x7]
  Product2/1 -> Ux/1
  xL/1 -> [xL]
  dX/1 -> [dX]
  S8/1 -> [S8]

== system RobustFormationControl_IntegerModel/Integer Leader and four followers/Follower 3 System/Follower 2 Quadrotor Model/Control Module1/Subsystem8 ==
  x3 : Inport
  x2 : Inport  Port=2
  x4 : Inport  Port=3
  x6 : Inport  Port=4
  xd3 : Inport  Port=5
  xd4 : Inport  Port=6
  S4 : Inport  Port=7
  Omega : Inport  Port=8
  Constant : Constant
  Constant3 : Constant  Value=d2
  Derivative : Derivative
  Divide : Product  Inputs=*/
  Product2 : Product
  Subsystem : Subsystem
  Subsystem1 : Subsystem
  Subsystem2 : Subsystem
  Sum2 : Sum  Inputs=+++
  U3 : Outport  VectorParamsAs1DForOutWhenUnconnected=off
  wires:
  Subsystem1/1(D1) -> Sum2/1
  Subsystem2/1(D3) -> Sum2/3
  Subsystem/1(D2) -> Sum2/2
  [xd4] -> Subsystem2/4(xd4)
  [x3] -> Subsystem2/1(x3)
  [x4] -> Subsystem2/3(x4)
  [S4] -> Subsystem2/5(S4)
  [xd3] -> Subsystem2/2(xd3)
  [S4] -> Subsystem/5(S4)
  [x4] -> Subsystem/3(x4)
  [xd4] -> Subsystem/4(xd4)
  [xd3] -> Subsystem/2(xd3)
  [xdDot4] -> Subsystem1/5(xd4)
  Omega/1 -> Subsystem1/4(Omega)
  [x2] -> Subsystem1/3(x2)
  [x6] -> Subsystem1/2(x6)
  [x4] -> Subsystem1/1(x4)
  [x3] -> Subsystem/1(x3)
  x3/1 -> [x3]
  x6/1 -> [x6]
  x4/1 -> [x4]
  Product2/1 -> U3/1
  Divide/1 -> Product2/1
  Sum2/1 -> Product2/2
  x2/1 -> [x2]
  xd3/1 -> [xd3]
  Derivative/1 -> [xdDot4]
  xd4/1 -> Derivative/1, [xd4]
  S4/1 -> [S4]
  Constant3/1 -> Divide/2
  Constant/1 -> Divide/1

== system RobustFormationControl_IntegerModel/Integer Leader and four followers/Follower 3 System/Follower 2 Quadrotor Model/Quadrotor Dynamic System/Rotational System ==
  U2 : Inport
  U3 : Inport  Port=2
  U4 : Inport  Port=3
  Omega : Inport  Port=4
  Equation1 : Subsystem
  Equation2 : Subsystem
  Equation3 : Subsystem
  Phi or x1 : Outport  VectorParamsAs1DForOutWhenUnconnected=off
  Theta or x3 : Outport  Port=2  VectorParamsAs1DForOutWhenUnconnected=off
  Psi or x5 : Outport  Port=3  VectorParamsAs1DForOutWhenUnconnected=off
  x2 : Outport  Port=4  VectorParamsAs1DForOutWhenUnconnected=off
  x4 : Outport  Port=5  VectorParamsAs1DForOutWhenUnconnected=off
  x6 : Outport  Port=6  VectorParamsAs1DForOutWhenUnconnected=off
  wires:
  Equation2/2(x4) -> Equation1/1(x4), Equation3/2(x4), x4/1
  Equation1/2(x2) -> Equation3/1(x2), Equation2/1(x2), x2/1
  Omega/1 -> Equation1/4(Omega), Equation2/4(Omega)
  U4/1 -> Equation3/3(U4)
  Equation2/1(x3 =Theta) -> Theta or x3/1
  Equation3/2(x6) -> Equation1/2(x6), x6/1, Equation2/2(x6)
  U3/1 -> Equation2/3(U3)
  U2/1 -> Equation1/3(U2)
  Equation3/1(x5 =Psi) -> Psi or x5/1
  Equation1/1(x1 = Phi) -> Phi or x1/1

== system RobustFormationControl_IntegerModel/Integer Leader and four followers/Follower 3 System/Follower 2 Quadrotor Model/Quadrotor Dynamic System/Translational System ==
  U1 : Inport
  Ux : Inport  Port=2
  Uy : Inport  Port=3
  x1 : Inport  Port=4
  x3 : Inport  Port=5
  Equation4 : Subsystem
  Equation5 : Subsystem
  Equation6 : Subsystem
  x or x7 : Outport  VectorParamsAs1DForOutWhenUnconnected=off
  y or x9 : Outport  Port=2  VectorParamsAs1DForOutWhenUnconnected=off
  z or x11 : Outport  Port=3  VectorParamsAs1DForOutWhenUnconnected=off
  xdot or x8 : Outport  Port=4  VectorParamsAs1DForOutWhenUnconnected=off
  ydot or x10 : Outport  Port=5  VectorParamsAs1DForOutWhenUnconnected=off
  zdot or x12 : Outport  Port=6  VectorParamsAs1DForOutWhenUnconnected=off
  wires:
  Equation6/2(x12 = zdot) -> zdot or x12/1
  Equation5/2(x10 = ydot) -> ydot or x10/1
  Equation4/2(x8 = xdot) -> xdot or x8/1
  U1/1 -> Equation4/1(U1), Equation5/1(U1), Equation6/1(U1)
  Equation4/1(x7 = x) -> x or x7/1
  Equation6/1(x11 = z) -> z or x11/1
  Equation5/1(x9 = y) -> y or x9/1
  x3/1 -> Equation6/3(x3)
  x1/1 -> Equation6/2(x1)
  Uy/1 -> Equation5/2(Uy)
  Ux/1 -> Equation4/2(Ux)

== system RobustFormationControl_IntegerModel/Integer Leader and four followers/Follower 4 System/Follower 2 Quadrotor Model/Control Module1/Desired System ==
  Phi_d : Inport
  Theta_d : Inport  Port=2
  Psi_d : Inport  Port=3
  xd : Inport  Port=4
  yd : Inport  Port=5
  zd : Inport  Port=6
  Derivative{,1..5} (6 alike) : Derivative
  xd1 : Outport  VectorParamsAs1DForOutWhenUnconnected=off
  xd2 : Outport  Port=2  VectorParamsAs1DForOutWhenUnconnected=off
  xd3 : Outport  Port=3  VectorParamsAs1DForOutWhenUnconnected=off
  xd4 : Outport  Port=4  VectorParamsAs1DForOutWhenUnconnected=off
  xd5 : Outport  Port=5  VectorParamsAs1DForOutWhenUnconnected=off
  xd6 : Outport  Port=6  VectorParamsAs1DForOutWhenUnconnected=off
  xd7 : Outport  Port=7  VectorParamsAs1DForOutWhenUnconnected=off
  xd8 : Outport  Port=8  VectorParamsAs1DForOutWhenUnconnected=off
  xd9 : Outport  Port=9  VectorParamsAs1DForOutWhenUnconnected=off
  xd10 : Outport  Port=10  VectorParamsAs1DForOutWhenUnconnected=off
  xd11 : Outport  Port=11  VectorParamsAs1DForOutWhenUnconnected=off
  xd12 : Outport  Port=12  VectorParamsAs1DForOutWhenUnconnected=off
  wires:
  Phi_d/1 -> Derivative/1, xd1/1
  Derivative/1 -> xd2/1
  Derivative1/1 -> xd4/1
  Theta_d/1 -> Derivative1/1, xd3/1
  Psi_d/1 -> Derivative2/1, xd5/1
  Derivative2/1 -> xd6/1
  Derivative3/1 -> xd8/1
  Derivative4/1 -> xd10/1
  Derivative5/1 -> xd12/1
  xd/1 -> Derivative3/1, xd7/1
  yd/1 -> Derivative4/1, xd9/1
  zd/1 -> Derivative5/1, xd11/1

== system RobustFormationControl_IntegerModel/Integer Leader and four followers/Follower 4 System/Follower 2 Quadrotor Model/Control Module1/Omega Equations ==
  U1 : Inport
  U2 : Inport  Port=2
  U3 : Inport  Port=3
  U4 : Inport  Port=4
  Add1 : Sum  Inputs=+--
  Add2 : Sum  Inputs=+++
  Add3 : Sum  Inputs=++-
  Add5 : Sum  Inputs=+-+
  Control Inputs : Subsystem
  Gain11 : Gain  Gain=1/(4*b)
  Gain12 : Gain  Gain=1/(4*d)
  Gain7 : Gain  Gain=1/(2*b)
  Gain8 : Gain  Gain=1/(2*b)
  Omega : Outport  VectorParamsAs1DForOutWhenUnconnected=off
  wires:
  Add5/1 -> Control Inputs/1(w1_sqt)
  Add1/1 -> Control Inputs/2(w2_sqt)
  Add2/1 -> Control Inputs/3(w3_sqt)
  Gain11/1 -> Add5/1, Add3/1, Add2/1, Add1/1
  Gain12/1 -> Add5/3, Add2/3, Add3/3, Add1/3
  Gain7/1 -> Add5/2, Add2/2
  Gain8/1 -> Add3/2, Add1/2
  U4/1 -> Gain12/1
  U1/1 -> Gain11/1
  U3/1 -> Gain7/1
  U2/1 -> Gain8/1
  Add3/1 -> Control Inputs/4(w4_sqt)
  Control Inputs/1(Omega) -> Omega/1

== system RobustFormationControl_IntegerModel/Integer Leader and four followers/Follower 4 System/Follower 2 Quadrotor Model/Control Module1/Subsystem ==
  Ux : Inport
  Uy : Inport  Port=2
  Psi_d : Inport  Port=3
  Subsystem : Subsystem
  Subsystem1 : Subsystem
  Phi_d : Outport  VectorParamsAs1DForOutWhenUnconnected=off
  Theta_d : Outport  Port=2  VectorParamsAs1DForOutWhenUnconnected=off
  wires:
  Ux/1 -> Subsystem1/1(Ux), Subsystem/1(Ux)
  Uy/1 -> Subsystem1/2(Uy), Subsystem/2(Uy)
  Psi_d/1 -> Subsystem1/3(Psi_d), Subsystem/3(Psi_d)
  Subsystem/1(Phi_d) -> Subsystem1/4(Phi_d), Phi_d/1
  Subsystem1/1(Theta_d) -> Theta_d/1

== system RobustFormationControl_IntegerModel/Integer Leader and four followers/Follower 4 System/Follower 2 Quadrotor Model/Control Module1/Subsystem1 ==
  x1 : Inport
  x2 : Inport  Port=2
  x3 : Inport  Port=3
  x4 : Inport  Port=4
  x5 : Inport  Port=5
  x6 : Inport  Port=6
  x7 : Inport  Port=7
  x8 : Inport  Port=8
  x9 : Inport  Port=9
  x10 : Inport  Port=10
  x11 : Inport  Port=11
  x12 : Inport  Port=12
  xd1 : Inport  Port=13
  xd2 : Inport  Port=14
  xd3 : Inport  Port=15
  xd4 : Inport  Port=16
  xd5 : Inport  Port=17
  xd6 : Inport  Port=18
  xL : Inport  Port=19
  dX : Inport  Port=20
  yL : Inport  Port=21
  dY : Inport  Port=22
  zL : Inport  Port=23
  dZ : Inport  Port=24
  Subsystem : Subsystem
  Subsystem1 : Subsystem
  Subsystem2 : Subsystem
  Subsystem3 : Subsystem
  Subsystem4 : Subsystem
  Subsystem6 : Subsystem
  S2 : Outport  VectorParamsAs1DForOutWhenUnconnected=off
  S4 : Outport  Port=2  VectorParamsAs1DForOutWhenUnconnected=off
  S6 : Outport  Port=3  VectorParamsAs1DForOutWhenUnconnected=off
  S8 : Outport  Port=4  VectorParamsAs1DForOutWhenUnconnected=off
  S10 : Outport  Port=5  VectorParamsAs1DForOutWhenUnconnected=off
  S12 : Outport  Port=6  VectorParamsAs1DForOutWhenUnconnected=off
  wires:
  x1/1 -> [x1]
  x2/1 -> [x2]
  x3/1 -> [x3]
  x4/1 -> [x4]
  x5/1 -> [x5]
  x6/1 -> [x6]
  x7/1 -> [x7]
  x8/1 -> [x8]
  x9/1 -> [x9]
  x10/1 -> [x10]
  x11/1 -> [x11]
  x12/1 -> [x12]
  xd1/1 -> [xd1]
  dY/1 -> [dY]
  xd2/1 -> [xd2]
  xd3/1 -> [xd3]
  xd4/1 -> [xd4]
  xd5/1 -> [xd5]
  xd6/1 -> [xd6]
  xL/1 -> [xL]
  dX/1 -> [dX]
  yL/1 -> [yL]
  zL/1 -> [zL]
  dZ/1 -> [dZ]
  [x1] -> Subsystem/1(x1)
  [xd1] -> Subsystem/2(xd1)
  [x2] -> Subsystem/3(x2)
  [xd2] -> Subsystem/4(xd2)
  Subsystem/1(S2) -> S2/1
  [xd4] -> Subsystem6/4(xd4)
  [x3] -> Subsystem6/1(x3)
  [x4] -> Subsystem6/3(x4)
  [xd3] -> Subsystem6/2(xd3)
  [xd6] -> Subsystem1/4(xd6)
  [x5] -> Subsystem1/1(x5)
  [x6] -> Subsystem1/3(x6)
  [xd5] -> Subsystem1/2(xd5)
  Subsystem6/1(S4) -> S4/1
  Subsystem1/1(S6) -> S6/1
  [x9] -> Subsystem2/2(x9)
  [x10] -> Subsystem2/3(x10)
  [yL] -> Subsystem2/1(yL)
  [dY] -> Subsystem2/4(dY)
  Subsystem2/1(S10) -> S10/1
  [zL] -> Subsystem4/1(zL)
  [x8] -> Subsystem3/3(x8)
  Subsystem4/1(S12) -> S12/1
  [x12] -> Subsystem4/3(x12)
  Subsystem3/1(S8) -> S8/1
  [dZ] -> Subsystem4/4(dZ)
  [x11] -> Subsystem4/2(x11)
  [x7] -> Subsystem3/2(x7)
  [dX] -> Subsystem3/4(dX)
  [xL] -> Subsystem3/1(xL)

== system RobustFormationControl_IntegerModel/Integer Leader and four followers/Follower 4 System/Follower 2 Quadrotor Model/Control Module1/Subsystem10 ==
  x1 : Inport
  x3 : Inport  Port=2
  x11 : Inport  Port=3
  x12 : Inport  Port=4
  zL : Inport  Port=5
  dZ : Inport  Port=6
  S12 : Inport  Port=7
  Constant1 : Constant
  Divide1 : Product  Inputs=*/
  Divide2 : Product  Inputs=**  RndMeth=Zero  SaturateOnIntegerOverflow=on
  Gain : Gain  Commented=on  Gain=b6
  Product1 : Product
  Product2 : Product
  Subsystem : Subsystem
  Subsystem1 : Subsystem
  Subsystem2 : Subsystem
  Sum2 : Sum  Inputs=+++
  Trigonometric Function1 : Trigonometry  Operator=cos
  Trigonometric Function2 : Trigonometry  Operator=cos
  U1 : Outport  VectorParamsAs1DForOutWhenUnconnected=off
  wires:
  S12/1 -> [S12]
  dZ/1 -> [dZ]
  zL/1 -> [zL]
  x3/1 -> [x3]
  Sum2/1 -> Product2/2
  Product2/1 -> U1/1
  x11/1 -> [x11]
  x12/1 -> [x12]
  x1/1 -> [x1]
  [x11] -> Subsystem/2(x11)
  [x12] -> Subsystem1/1(x12)
  [zL] -> Subsystem1/2(zL)
  [zL] -> Subsystem/1(zL)
  [dZ] -> Subsystem/4(dZ)
  [x12] -> Subsystem/3(x12)
  [S12] -> Subsystem/5(S12)
  [x11] -> Subsystem2/2(x11)
  [S12] -> Subsystem2/5(S12)
  [x12] -> Subsystem2/3(x12)
  [zL] -> Subsystem2/1(zL)
  [dZ] -> Subsystem2/4(dZ)
  Subsystem/1(D2) -> Sum2/2
  Subsystem2/1(D3) -> Sum2/3
  Subsystem1/1(D1) -> Sum2/1
  Divide1/1 -> Product2/1
  Constant1/1 -> Divide1/1
  Trigonometric Function2/1 -> Product1/2
  Trigonometric Function1/1 -> Product1/1
  Divide2/1 -> Divide1/2
  Product1/1 -> Divide2/2
  [x1] -> Trigonometric Function1/1
  [x3] -> Trigonometric Function2/1
  [b6D] -> Divide2/1
  [dZ] -> Subsystem1/3(dZ)

== system RobustFormationControl_IntegerModel/Integer Leader and four followers/Follower 4 System/Follower 2 Quadrotor Model/Control Module1/Subsystem2 ==
  U1 : Inport
  x9 : Inport  Port=2
  x10 : Inport  Port=3
  yL : Inport  Port=4
  dY : Inport  Port=5
  S10 : Inport  Port=6
  Constant1 : Constant
  Divide1 : Product  Inputs=*/
  Divide2 : Product  Inputs=**  RndMeth=Zero  SaturateOnIntegerOverflow=on
  Gain1 : Gain  Commented=on  Gain=b4
  Product2 : Product
  Subsystem3 : Subsystem
  Subsystem4 : Subsystem
  Subsystem5 : Subsystem
  Sum1 : Sum  Inputs=+++
  Uy : Outport  VectorParamsAs1DForOutWhenUnconnected=off
  wires:
  S10/1 -> [S10]
  dY/1 -> [dY]
  yL/1 -> [yL]
  Product2/1 -> Uy/1
  x9/1 -> [x9]
  x10/1 -> [x10]
  U1/1 -> [U1]
  Divide1/1 -> Product2/1
  Constant1/1 -> Divide1/1
  [b5D] -> Divide2/1
  [U1] -> Divide2/2
  Divide2/1 -> Divide1/2
  [dY] -> Subsystem4/3(dY)
  [dY] -> Subsystem3/4(dY)
  Subsystem4/1(D1) -> Sum1/1
  Subsystem5/1(D3) -> Sum1/3
  [yL] -> Subsystem5/1(yL)
  Subsystem3/1(D2) -> Sum1/2
  [dY] -> Subsystem5/4(dY)
  [x9] -> Subsystem3/2(x9)
  [yL] -> Subsystem3/1(yL)
  [yL] -> Subsystem4/2(yL)
  [S10] -> Subsystem3/5(S10)
  [x9] -> Subsystem5/2(x9)
  [x10] -> Subsystem5/3(x10)
  [x10] -> Subsystem4/1(x10)
  [x10] -> Subsystem3/3(x10)
  [S10] -> Subsystem5/5(S10)
  Sum1/1 -> Product2/2

== system RobustFormationControl_IntegerModel/Integer Leader and four followers/Follower 4 System/Follower 2 Quadrotor Model/Control Module1/Subsystem4 ==
  x1 : Inport
  x2 : Inport  Port=2
  x4 : Inport  Port=3
  x6 : Inport  Port=4
  xd1 : Inport  Port=5
  xd2 : Inport  Port=6
  S2 : Inport  Port=7
  Omega : Inport  Port=8
  Constant : Constant
  Constant3 : Constant  Value=d1
  Derivative : Derivative
  Divide : Product  Inputs=*/
  Product2 : Product
  Subsystem : Subsystem
  Subsystem1 : Subsystem
  Subsystem2 : Subsystem
  Sum2 : Sum  Inputs=+++
  U2 : Outport  VectorParamsAs1DForOutWhenUnconnected=off
  wires:
  Constant/1 -> Divide/1
  Constant3/1 -> Divide/2
  S2/1 -> [S2]
  xd2/1 -> [xd2], Derivative/1
  Derivative/1 -> [xdDot2]
  xd1/1 -> [xd1]
  x2/1 -> [x2]
  Sum2/1 -> Product2/2
  Divide/1 -> Product2/1
  Product2/1 -> U2/1
  x4/1 -> [x4]
  x6/1 -> [x6]
  x1/1 -> [x1]
  [x1] -> Subsystem/1(x1)
  [x4] -> Subsystem1/1(x4)
  [x6] -> Subsystem1/2(x6)
  [x2] -> Subsystem1/3(x2)
  Omega/1 -> Subsystem1/4(Omega)
  [xdDot2] -> Subsystem1/5(xd2)
  [xd1] -> Subsystem/2(xd1)
  [xd2] -> Subsystem/4(xd2)
  [x2] -> Subsystem/3(x2)
  [S2] -> Subsystem/5(S2)
  [xd1] -> Subsystem2/2(xd1)
  [S2] -> Subsystem2/5(S2)
  [x2] -> Subsystem2/3(x2)
  [x1] -> Subsystem2/1(x1)
  [xd2] -> Subsystem2/4(xd2)
  Subsystem1/1(D1) -> Sum2/1
  Subsystem/1(D2) -> Sum2/2
  Subsystem2/1(D3) -> Sum2/3

== system RobustFormationControl_IntegerModel/Integer Leader and four followers/Follower 4 System/Follower 2 Quadrotor Model/Control Module1/Subsystem5 ==
  x5 : Inport
  x2 : Inport  Port=2
  x4 : Inport  Port=3
  x6 : Inport  Port=4
  xd5 : Inport  Port=5
  xd6 : Inport  Port=6
  S6 : Inport  Port=7
  Constant : Constant
  Constant3 : Constant  Value=c3
  Derivative : Derivative
  Divide : Product  Inputs=*/
  Product2 : Product
  Subsystem : Subsystem
  Subsystem1 : Subsystem
  Subsystem2 : Subsystem
  Sum2 : Sum  Inputs=+++
  U4 : Outport  VectorParamsAs1DForOutWhenUnconnected=off
  wires:
  Constant/1 -> Divide/1
  Constant3/1 -> Divide/2
  S6/1 -> [S6]
  xd6/1 -> [xd6], Derivative/1
  Derivative/1 -> [xdDot6]
  xd5/1 -> [xd5]
  x2/1 -> [x2]
  Sum2/1 -> Product2/2
  Divide/1 -> Product2/1
  Product2/1 -> U4/1
  x4/1 -> [x4]
  x6/1 -> [x6]
  x5/1 -> [x5]
  [x5] -> Subsystem/1(x5)
  [x4] -> Subsystem1/1(x4)
  [x6] -> Subsystem1/2(x6)
  [x2] -> Subsystem1/3(x2)
  [xdDot6] -> Subsystem1/4(xd6)
  [xd5] -> Subsystem/2(xd5)
  [xd6] -> Subsystem/4(xd6)
  [x6] -> Subsystem/3(x6)
  [S6] -> Subsystem/5(S4)
  [xd5] -> Subsystem2/2(xd5)
  [S6] -> Subsystem2/5(S6)
  [x6] -> Subsystem2/3(x6)
  [x5] -> Subsystem2/1(x5)
  [xd6] -> Subsystem2/4(xd6)
  Subsystem/1(D2) -> Sum2/2
  Subsystem2/1(D3) -> Sum2/3
  Subsystem1/1(D1) -> Sum2/1
